simulink model "testTSTop"  (R2026a)
settings: Solver=FixedStepDiscrete  FixedStep=0.1
settings Model: Creator=grouleau  LastModifiedBy=grouleau

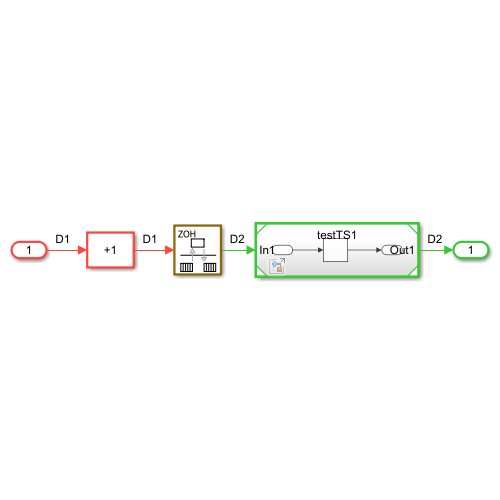
[thumbnail: Simulink's stored preview of the top-level diagram]
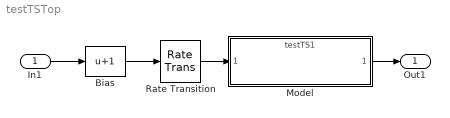
== system testTSTop ==
  In1 : Inport  SampleTime=0.1
  Bias : Bias  Bias=1  SaturateOnIntegerOverflow=off
  Model : ModelReference  ModelNameDialog=testTS1  SimulationMode=Normal  ModelReferenceVersion=1.3
  Rate Transition : RateTransition
  Out1 : Outport
  wires:
  In1/1 -> Bias/1
  Bias/1 -> Rate Transition/1
  Model/1 -> Out1/1
  Rate Transition/1 -> Model/1
